simulink library "lib_SecCtrl_MASmsg"  (R2026a)
settings: Solver=VariableStepAuto
undefined symbols (not defined in the file): buses_lf, DiscIntNeverNeededParam, entity, iPs_lf, iQs_lf, last_send, m, Ps_lf, Qs_lf, set_DG_up, set_extra_satur, set_sending_cost, v_buses_mod
libraries: simulink x400, sl_discontinuities x10, eeGeneralControl x5
(part 12 of 12)

== system lib_SecCtrl_MASmsg/MAS messages/ID3/Send to neighbor1/one/select ==
  select : TriggerPort  TriggerType=function-call  IsSimulinkFunction=on  FunctionName=select  FunctionVisibility=scoped  VariantControl=(inherit)
  All : simulink/Logic and Bit Operations/Compare To Constant  relop===  const=0  OutDataTypeStr=boolean  ZeroCross=off
  Gain : Gain  OutDataTypeStr=double
  Gain2 : Gain  Gain=2  OutDataTypeStr=double
  Neighbor : simulink/Logic and Bit Operations/Compare To Constant  relop===  const=2  OutDataTypeStr=boolean  ZeroCross=off
  Sum : Sum  Inputs=|++
  u : ArgIn  DisableCoverage=on  ArgumentName=u
  y : ArgOut  ArgumentName=y
  wires:
  u/1 -> All/1, Neighbor/1
  Neighbor/1 -> Gain/1
  Gain2/1 -> Sum/2
  All/1 -> Gain2/1
  Sum/1 -> y/1
  Gain/1 -> Sum/1

== system lib_SecCtrl_MASmsg/MAS messages/ID3/Send to neighbor1/three/select ==
  select : TriggerPort  TriggerType=function-call  IsSimulinkFunction=on  FunctionName=select  FunctionVisibility=scoped  VariantControl=(inherit)
  All : simulink/Logic and Bit Operations/Compare To Constant  relop===  const=0  OutDataTypeStr=boolean  ZeroCross=off
  Gain : Gain  OutDataTypeStr=double
  Gain1 : Gain  Gain=2  OutDataTypeStr=double
  Gain2 : Gain  Gain=4  OutDataTypeStr=double
  Gain3 : Gain  Gain=3  OutDataTypeStr=double
  Neighbor1 : simulink/Logic and Bit Operations/Compare To Constant  relop===  const=0  OutDataTypeStr=boolean  ZeroCross=off
  Neighbor2 : simulink/Logic and Bit Operations/Compare To Constant  relop===  const=0  OutDataTypeStr=boolean  ZeroCross=off
  Neighbor3 : simulink/Logic and Bit Operations/Compare To Constant  relop===  const=0  OutDataTypeStr=boolean  ZeroCross=off
  Sum : Sum  Inputs=|++++
  u : ArgIn  DisableCoverage=on  ArgumentName=u
  y : ArgOut  ArgumentName=y
  wires:
  Neighbor2/1 -> Gain1/1
  u/1 -> Neighbor3/1, All/1, Neighbor1/1, Neighbor2/1
  Neighbor1/1 -> Gain/1
  Gain2/1 -> Sum/4
  All/1 -> Gain2/1
  Gain1/1 -> Sum/2
  Sum/1 -> y/1
  Gain/1 -> Sum/1
  Neighbor3/1 -> Gain3/1
  Gain3/1 -> Sum/3

== system lib_SecCtrl_MASmsg/MAS messages/ID3/Send to neighbor1/two/select ==
  select : TriggerPort  TriggerType=function-call  IsSimulinkFunction=on  FunctionName=select  FunctionVisibility=scoped  VariantControl=(inherit)
  All : simulink/Logic and Bit Operations/Compare To Constant  relop===  const=0  OutDataTypeStr=boolean  ZeroCross=off
  Gain : Gain  OutDataTypeStr=double
  Gain1 : Gain  Gain=2  OutDataTypeStr=double
  Gain2 : Gain  Gain=3  OutDataTypeStr=double
  Neighbor1 : simulink/Logic and Bit Operations/Compare To Constant  relop===  const=2  OutDataTypeStr=boolean  ZeroCross=off
  Neighbor2 : simulink/Logic and Bit Operations/Compare To Constant  relop===  const=4  OutDataTypeStr=boolean  ZeroCross=off
  Sum : Sum  Inputs=|+++
  u : ArgIn  DisableCoverage=on  ArgumentName=u
  y : ArgOut  ArgumentName=y
  wires:
  Neighbor2/1 -> Gain1/1
  u/1 -> All/1, Neighbor1/1, Neighbor2/1
  Neighbor1/1 -> Gain/1
  Gain2/1 -> Sum/3
  All/1 -> Gain2/1
  Gain1/1 -> Sum/2
  Sum/1 -> y/1
  Gain/1 -> Sum/1

== system lib_SecCtrl_MASmsg/MAS messages/ID3/Send to neighbor2/five/select ==
  select : TriggerPort  TriggerType=function-call  IsSimulinkFunction=on  FunctionName=select  FunctionVisibility=scoped  VariantControl=(inherit)
  All : simulink/Logic and Bit Operations/Compare To Constant  relop===  const=0  OutDataTypeStr=boolean  ZeroCross=off
  Gain : Gain  OutDataTypeStr=double
  Gain1 : Gain  Gain=2  OutDataTypeStr=double
  Gain2 : Gain  Gain=6  OutDataTypeStr=double
  Gain3 : Gain  Gain=3  OutDataTypeStr=double
  Gain4 : Gain  Gain=4  OutDataTypeStr=double
  Gain5 : Gain  Gain=5  OutDataTypeStr=double
  Neighbor1 : simulink/Logic and Bit Operations/Compare To Constant  relop===  const=2  OutDataTypeStr=boolean  ZeroCross=off
  Neighbor2 : simulink/Logic and Bit Operations/Compare To Constant  relop===  const=2  OutDataTypeStr=boolean  ZeroCross=off
  Neighbor3 : simulink/Logic and Bit Operations/Compare To Constant  relop===  const=0  OutDataTypeStr=boolean  ZeroCross=off
  Neighbor4 : simulink/Logic and Bit Operations/Compare To Constant  relop===  const=0  OutDataTypeStr=boolean  ZeroCross=off
  Neighbor5 : simulink/Logic and Bit Operations/Compare To Constant  relop===  const=0  OutDataTypeStr=boolean  ZeroCross=off
  Sum : Sum  Inputs=|++++++
  u : ArgIn  DisableCoverage=on  ArgumentName=u
  y : ArgOut  ArgumentName=y
  wires:
  Neighbor5/1 -> Gain5/1
  Gain5/1 -> Sum/5
  Neighbor2/1 -> Gain1/1
  u/1 -> Neighbor3/1, Neighbor4/1, All/1, Neighbor5/1, Neighbor1/1, Neighbor2/1
  Neighbor1/1 -> Gain/1
  Gain2/1 -> Sum/6
  All/1 -> Gain2/1
  Gain1/1 -> Sum/2
  Sum/1 -> y/1
  Gain/1 -> Sum/1
  Neighbor3/1 -> Gain3/1
  Gain3/1 -> Sum/3
  Gain4/1 -> Sum/4
  Neighbor4/1 -> Gain4/1

== system lib_SecCtrl_MASmsg/MAS messages/ID3/Send to neighbor2/four/select ==
  select : TriggerPort  TriggerType=function-call  IsSimulinkFunction=on  FunctionName=select  FunctionVisibility=scoped  VariantControl=(inherit)
  All : simulink/Logic and Bit Operations/Compare To Constant  relop===  const=0  OutDataTypeStr=boolean  ZeroCross=off
  Gain : Gain  OutDataTypeStr=double
  Gain1 : Gain  Gain=2  OutDataTypeStr=double
  Gain2 : Gain  Gain=5  OutDataTypeStr=double
  Gain3 : Gain  Gain=3  OutDataTypeStr=double
  Gain4 : Gain  Gain=4  OutDataTypeStr=double
  Neighbor1 : simulink/Logic and Bit Operations/Compare To Constant  relop===  const=1  OutDataTypeStr=boolean  ZeroCross=off
  Neighbor2 : simulink/Logic and Bit Operations/Compare To Constant  relop===  const=3  OutDataTypeStr=boolean  ZeroCross=off
  Neighbor3 : simulink/Logic and Bit Operations/Compare To Constant  relop===  const=0  OutDataTypeStr=boolean  ZeroCross=off
  Neighbor4 : simulink/Logic and Bit Operations/Compare To Constant  relop===  const=0  OutDataTypeStr=boolean  ZeroCross=off
  Sum : Sum  Inputs=|+++++
  u : ArgIn  DisableCoverage=on  ArgumentName=u
  y : ArgOut  ArgumentName=y
  wires:
  Neighbor4/1 -> Gain4/1
  Gain4/1 -> Sum/4
  Gain3/1 -> Sum/3
  Neighbor3/1 -> Gain3/1
  Gain/1 -> Sum/1
  Sum/1 -> y/1
  Gain1/1 -> Sum/2
  All/1 -> Gain2/1
  Gain2/1 -> Sum/5
  Neighbor1/1 -> Gain/1
  u/1 -> Neighbor2/1, Neighbor1/1, All/1, Neighbor4/1, Neighbor3/1
  Neighbor2/1 -> Gain1/1

== system lib_SecCtrl_MASmsg/MAS messages/ID3/Send to neighbor2/one/select ==
  select : TriggerPort  TriggerType=function-call  IsSimulinkFunction=on  FunctionName=select  FunctionVisibility=scoped  VariantControl=(inherit)
  All : simulink/Logic and Bit Operations/Compare To Constant  relop===  const=0  OutDataTypeStr=boolean  ZeroCross=off
  Gain : Gain  OutDataTypeStr=double
  Gain2 : Gain  Gain=2  OutDataTypeStr=double
  Neighbor : simulink/Logic and Bit Operations/Compare To Constant  relop===  const=2  OutDataTypeStr=boolean  ZeroCross=off
  Sum : Sum  Inputs=|++
  u : ArgIn  DisableCoverage=on  ArgumentName=u
  y : ArgOut  ArgumentName=y
  wires:
  Gain/1 -> Sum/1
  Sum/1 -> y/1
  All/1 -> Gain2/1
  Gain2/1 -> Sum/2
  Neighbor/1 -> Gain/1
  u/1 -> Neighbor/1, All/1

== system lib_SecCtrl_MASmsg/MAS messages/ID3/Send to neighbor2/three/select ==
  select : TriggerPort  TriggerType=function-call  IsSimulinkFunction=on  FunctionName=select  FunctionVisibility=scoped  VariantControl=(inherit)
  All : simulink/Logic and Bit Operations/Compare To Constant  relop===  const=0  OutDataTypeStr=boolean  ZeroCross=off
  Gain : Gain  OutDataTypeStr=double
  Gain1 : Gain  Gain=2  OutDataTypeStr=double
  Gain2 : Gain  Gain=4  OutDataTypeStr=double
  Gain3 : Gain  Gain=3  OutDataTypeStr=double
  Neighbor1 : simulink/Logic and Bit Operations/Compare To Constant  relop===  const=0  OutDataTypeStr=boolean  ZeroCross=off
  Neighbor2 : simulink/Logic and Bit Operations/Compare To Constant  relop===  const=0  OutDataTypeStr=boolean  ZeroCross=off
  Neighbor3 : simulink/Logic and Bit Operations/Compare To Constant  relop===  const=0  OutDataTypeStr=boolean  ZeroCross=off
  Sum : Sum  Inputs=|++++
  u : ArgIn  DisableCoverage=on  ArgumentName=u
  y : ArgOut  ArgumentName=y
  wires:
  Gain3/1 -> Sum/3
  Neighbor3/1 -> Gain3/1
  Gain/1 -> Sum/1
  Sum/1 -> y/1
  Gain1/1 -> Sum/2
  All/1 -> Gain2/1
  Gain2/1 -> Sum/4
  Neighbor1/1 -> Gain/1
  u/1 -> Neighbor2/1, Neighbor1/1, All/1, Neighbor3/1
  Neighbor2/1 -> Gain1/1

== system lib_SecCtrl_MASmsg/MAS messages/ID3/Send to neighbor2/two/select ==
  select : TriggerPort  TriggerType=function-call  IsSimulinkFunction=on  FunctionName=select  FunctionVisibility=scoped  VariantControl=(inherit)
  All : simulink/Logic and Bit Operations/Compare To Constant  relop===  const=0  OutDataTypeStr=boolean  ZeroCross=off
  Gain : Gain  OutDataTypeStr=double
  Gain1 : Gain  Gain=2  OutDataTypeStr=double
  Gain2 : Gain  Gain=3  OutDataTypeStr=double
  Neighbor1 : simulink/Logic and Bit Operations/Compare To Constant  relop===  const=2  OutDataTypeStr=boolean  ZeroCross=off
  Neighbor2 : simulink/Logic and Bit Operations/Compare To Constant  relop===  const=4  OutDataTypeStr=boolean  ZeroCross=off
  Sum : Sum  Inputs=|+++
  u : ArgIn  DisableCoverage=on  ArgumentName=u
  y : ArgOut  ArgumentName=y
  wires:
  Gain/1 -> Sum/1
  Sum/1 -> y/1
  Gain1/1 -> Sum/2
  All/1 -> Gain2/1
  Gain2/1 -> Sum/3
  Neighbor1/1 -> Gain/1
  u/1 -> Neighbor2/1, Neighbor1/1, All/1
  Neighbor2/1 -> Gain1/1

== system lib_SecCtrl_MASmsg/MAS messages/ID4/Send to neighbor/five/select ==
  select : TriggerPort  TriggerType=function-call  IsSimulinkFunction=on  FunctionName=select  FunctionVisibility=scoped  VariantControl=(inherit)
  All : simulink/Logic and Bit Operations/Compare To Constant  relop===  const=0  OutDataTypeStr=boolean  ZeroCross=off
  Gain : Gain  OutDataTypeStr=double
  Gain1 : Gain  Gain=2  OutDataTypeStr=double
  Gain2 : Gain  Gain=6  OutDataTypeStr=double
  Gain3 : Gain  Gain=3  OutDataTypeStr=double
  Gain4 : Gain  Gain=4  OutDataTypeStr=double
  Gain5 : Gain  Gain=5  OutDataTypeStr=double
  Neighbor1 : simulink/Logic and Bit Operations/Compare To Constant  relop===  const=2  OutDataTypeStr=boolean  ZeroCross=off
  Neighbor2 : simulink/Logic and Bit Operations/Compare To Constant  relop===  const=2  OutDataTypeStr=boolean  ZeroCross=off
  Neighbor3 : simulink/Logic and Bit Operations/Compare To Constant  relop===  const=0  OutDataTypeStr=boolean  ZeroCross=off
  Neighbor4 : simulink/Logic and Bit Operations/Compare To Constant  relop===  const=0  OutDataTypeStr=boolean  ZeroCross=off
  Neighbor5 : simulink/Logic and Bit Operations/Compare To Constant  relop===  const=0  OutDataTypeStr=boolean  ZeroCross=off
  Sum : Sum  Inputs=|++++++
  u : ArgIn  DisableCoverage=on  ArgumentName=u
  y : ArgOut  ArgumentName=y
  wires:
  Neighbor5/1 -> Gain5/1
  Gain5/1 -> Sum/5
  Neighbor2/1 -> Gain1/1
  u/1 -> Neighbor3/1, Neighbor4/1, All/1, Neighbor5/1, Neighbor1/1, Neighbor2/1
  Neighbor1/1 -> Gain/1
  Gain2/1 -> Sum/6
  All/1 -> Gain2/1
  Gain1/1 -> Sum/2
  Sum/1 -> y/1
  Gain/1 -> Sum/1
  Neighbor3/1 -> Gain3/1
  Gain3/1 -> Sum/3
  Gain4/1 -> Sum/4
  Neighbor4/1 -> Gain4/1

== system lib_SecCtrl_MASmsg/MAS messages/ID4/Send to neighbor/four/select ==
  select : TriggerPort  TriggerType=function-call  IsSimulinkFunction=on  FunctionName=select  FunctionVisibility=scoped  VariantControl=(inherit)
  All : simulink/Logic and Bit Operations/Compare To Constant  relop===  const=0  OutDataTypeStr=boolean  ZeroCross=off
  Gain : Gain  OutDataTypeStr=double
  Gain1 : Gain  Gain=2  OutDataTypeStr=double
  Gain2 : Gain  Gain=5  OutDataTypeStr=double
  Gain3 : Gain  Gain=3  OutDataTypeStr=double
  Gain4 : Gain  Gain=4  OutDataTypeStr=double
  Neighbor1 : simulink/Logic and Bit Operations/Compare To Constant  relop===  const=1  OutDataTypeStr=boolean  ZeroCross=off
  Neighbor2 : simulink/Logic and Bit Operations/Compare To Constant  relop===  const=3  OutDataTypeStr=boolean  ZeroCross=off
  Neighbor3 : simulink/Logic and Bit Operations/Compare To Constant  relop===  const=0  OutDataTypeStr=boolean  ZeroCross=off
  Neighbor4 : simulink/Logic and Bit Operations/Compare To Constant  relop===  const=0  OutDataTypeStr=boolean  ZeroCross=off
  Sum : Sum  Inputs=|+++++
  u : ArgIn  DisableCoverage=on  ArgumentName=u
  y : ArgOut  ArgumentName=y
  wires:
  Neighbor4/1 -> Gain4/1
  Gain4/1 -> Sum/4
  Gain3/1 -> Sum/3
  Neighbor3/1 -> Gain3/1
  Gain/1 -> Sum/1
  Sum/1 -> y/1
  Gain1/1 -> Sum/2
  All/1 -> Gain2/1
  Gain2/1 -> Sum/5
  Neighbor1/1 -> Gain/1
  u/1 -> Neighbor2/1, Neighbor1/1, All/1, Neighbor4/1, Neighbor3/1
  Neighbor2/1 -> Gain1/1

== system lib_SecCtrl_MASmsg/MAS messages/ID4/Send to neighbor/one/select ==
  select : TriggerPort  TriggerType=function-call  IsSimulinkFunction=on  FunctionName=select  FunctionVisibility=scoped  VariantControl=(inherit)
  All : simulink/Logic and Bit Operations/Compare To Constant  relop===  const=0  OutDataTypeStr=boolean  ZeroCross=off
  Gain : Gain  OutDataTypeStr=double
  Gain2 : Gain  Gain=2  OutDataTypeStr=double
  Neighbor : simulink/Logic and Bit Operations/Compare To Constant  relop===  const=2  OutDataTypeStr=boolean  ZeroCross=off
  Sum : Sum  Inputs=|++
  u : ArgIn  DisableCoverage=on  ArgumentName=u
  y : ArgOut  ArgumentName=y
  wires:
  Gain/1 -> Sum/1
  Sum/1 -> y/1
  All/1 -> Gain2/1
  Gain2/1 -> Sum/2
  Neighbor/1 -> Gain/1
  u/1 -> Neighbor/1, All/1

== system lib_SecCtrl_MASmsg/MAS messages/ID4/Send to neighbor/three/select ==
  select : TriggerPort  TriggerType=function-call  IsSimulinkFunction=on  FunctionName=select  FunctionVisibility=scoped  VariantControl=(inherit)
  All : simulink/Logic and Bit Operations/Compare To Constant  relop===  const=0  OutDataTypeStr=boolean  ZeroCross=off
  Gain : Gain  OutDataTypeStr=double
  Gain1 : Gain  Gain=2  OutDataTypeStr=double
  Gain2 : Gain  Gain=4  OutDataTypeStr=double
  Gain3 : Gain  Gain=3  OutDataTypeStr=double
  Neighbor1 : simulink/Logic and Bit Operations/Compare To Constant  relop===  const=0  OutDataTypeStr=boolean  ZeroCross=off
  Neighbor2 : simulink/Logic and Bit Operations/Compare To Constant  relop===  const=0  OutDataTypeStr=boolean  ZeroCross=off
  Neighbor3 : simulink/Logic and Bit Operations/Compare To Constant  relop===  const=0  OutDataTypeStr=boolean  ZeroCross=off
  Sum : Sum  Inputs=|++++
  u : ArgIn  DisableCoverage=on  ArgumentName=u
  y : ArgOut  ArgumentName=y
  wires:
  Gain3/1 -> Sum/3
  Neighbor3/1 -> Gain3/1
  Gain/1 -> Sum/1
  Sum/1 -> y/1
  Gain1/1 -> Sum/2
  All/1 -> Gain2/1
  Gain2/1 -> Sum/4
  Neighbor1/1 -> Gain/1
  u/1 -> Neighbor2/1, Neighbor1/1, All/1, Neighbor3/1
  Neighbor2/1 -> Gain1/1

== system lib_SecCtrl_MASmsg/MAS messages/ID4/Send to neighbor/two/select ==
  select : TriggerPort  TriggerType=function-call  IsSimulinkFunction=on  FunctionName=select  FunctionVisibility=scoped  VariantControl=(inherit)
  All : simulink/Logic and Bit Operations/Compare To Constant  relop===  const=0  OutDataTypeStr=boolean  ZeroCross=off
  Gain : Gain  OutDataTypeStr=double
  Gain1 : Gain  Gain=2  OutDataTypeStr=double
  Gain2 : Gain  Gain=3  OutDataTypeStr=double
  Neighbor1 : simulink/Logic and Bit Operations/Compare To Constant  relop===  const=3  OutDataTypeStr=boolean  ZeroCross=off
  Neighbor2 : simulink/Logic and Bit Operations/Compare To Constant  relop===  const=5  OutDataTypeStr=boolean  ZeroCross=off
  Sum : Sum  Inputs=|+++
  u : ArgIn  DisableCoverage=on  ArgumentName=u
  y : ArgOut  ArgumentName=y
  wires:
  Gain/1 -> Sum/1
  Sum/1 -> y/1
  Gain1/1 -> Sum/2
  All/1 -> Gain2/1
  Gain2/1 -> Sum/3
  Neighbor1/1 -> Gain/1
  u/1 -> Neighbor2/1, Neighbor1/1, All/1
  Neighbor2/1 -> Gain1/1

== system lib_SecCtrl_MASmsg/MAS messages/ID4/Send to neighbor1/five/select ==
  select : TriggerPort  TriggerType=function-call  IsSimulinkFunction=on  FunctionName=select  FunctionVisibility=scoped  VariantControl=(inherit)
  All : simulink/Logic and Bit Operations/Compare To Constant  relop===  const=0  OutDataTypeStr=boolean  ZeroCross=off
  Gain : Gain  OutDataTypeStr=double
  Gain1 : Gain  Gain=2  OutDataTypeStr=double
  Gain2 : Gain  Gain=6  OutDataTypeStr=double
  Gain3 : Gain  Gain=3  OutDataTypeStr=double
  Gain4 : Gain  Gain=4  OutDataTypeStr=double
  Gain5 : Gain  Gain=5  OutDataTypeStr=double
  Neighbor1 : simulink/Logic and Bit Operations/Compare To Constant  relop===  const=2  OutDataTypeStr=boolean  ZeroCross=off
  Neighbor2 : simulink/Logic and Bit Operations/Compare To Constant  relop===  const=2  OutDataTypeStr=boolean  ZeroCross=off
  Neighbor3 : simulink/Logic and Bit Operations/Compare To Constant  relop===  const=0  OutDataTypeStr=boolean  ZeroCross=off
  Neighbor4 : simulink/Logic and Bit Operations/Compare To Constant  relop===  const=0  OutDataTypeStr=boolean  ZeroCross=off
  Neighbor5 : simulink/Logic and Bit Operations/Compare To Constant  relop===  const=0  OutDataTypeStr=boolean  ZeroCross=off
  Sum : Sum  Inputs=|++++++
  u : ArgIn  DisableCoverage=on  ArgumentName=u
  y : ArgOut  ArgumentName=y
  wires:
  Neighbor4/1 -> Gain4/1
  Gain4/1 -> Sum/4
  Gain3/1 -> Sum/3
  Neighbor3/1 -> Gain3/1
  Gain/1 -> Sum/1
  Sum/1 -> y/1
  Gain1/1 -> Sum/2
  All/1 -> Gain2/1
  Gain2/1 -> Sum/6
  Neighbor1/1 -> Gain/1
  u/1 -> Neighbor2/1, Neighbor1/1, Neighbor5/1, All/1, Neighbor4/1, Neighbor3/1
  Neighbor2/1 -> Gain1/1
  Gain5/1 -> Sum/5
  Neighbor5/1 -> Gain5/1

== system lib_SecCtrl_MASmsg/MAS messages/ID4/Send to neighbor1/four/select ==
  select : TriggerPort  TriggerType=function-call  IsSimulinkFunction=on  FunctionName=select  FunctionVisibility=scoped  VariantControl=(inherit)
  All : simulink/Logic and Bit Operations/Compare To Constant  relop===  const=0  OutDataTypeStr=boolean  ZeroCross=off
  Gain : Gain  OutDataTypeStr=double
  Gain1 : Gain  Gain=2  OutDataTypeStr=double
  Gain2 : Gain  Gain=5  OutDataTypeStr=double
  Gain3 : Gain  Gain=3  OutDataTypeStr=double
  Gain4 : Gain  Gain=4  OutDataTypeStr=double
  Neighbor1 : simulink/Logic and Bit Operations/Compare To Constant  relop===  const=1  OutDataTypeStr=boolean  ZeroCross=off
  Neighbor2 : simulink/Logic and Bit Operations/Compare To Constant  relop===  const=3  OutDataTypeStr=boolean  ZeroCross=off
  Neighbor3 : simulink/Logic and Bit Operations/Compare To Constant  relop===  const=0  OutDataTypeStr=boolean  ZeroCross=off
  Neighbor4 : simulink/Logic and Bit Operations/Compare To Constant  relop===  const=0  OutDataTypeStr=boolean  ZeroCross=off
  Sum : Sum  Inputs=|+++++
  u : ArgIn  DisableCoverage=on  ArgumentName=u
  y : ArgOut  ArgumentName=y
  wires:
  Neighbor2/1 -> Gain1/1
  u/1 -> Neighbor3/1, Neighbor4/1, All/1, Neighbor1/1, Neighbor2/1
  Neighbor1/1 -> Gain/1
  Gain2/1 -> Sum/5
  All/1 -> Gain2/1
  Gain1/1 -> Sum/2
  Sum/1 -> y/1
  Gain/1 -> Sum/1
  Neighbor3/1 -> Gain3/1
  Gain3/1 -> Sum/3
  Gain4/1 -> Sum/4
  Neighbor4/1 -> Gain4/1

== system lib_SecCtrl_MASmsg/MAS messages/ID4/Send to neighbor1/one/select ==
  select : TriggerPort  TriggerType=function-call  IsSimulinkFunction=on  FunctionName=select  FunctionVisibility=scoped  VariantControl=(inherit)
  All : simulink/Logic and Bit Operations/Compare To Constant  relop===  const=0  OutDataTypeStr=boolean  ZeroCross=off
  Gain : Gain  OutDataTypeStr=double
  Gain2 : Gain  Gain=2  OutDataTypeStr=double
  Neighbor : simulink/Logic and Bit Operations/Compare To Constant  relop===  const=2  OutDataTypeStr=boolean  ZeroCross=off
  Sum : Sum  Inputs=|++
  u : ArgIn  DisableCoverage=on  ArgumentName=u
  y : ArgOut  ArgumentName=y
  wires:
  u/1 -> All/1, Neighbor/1
  Neighbor/1 -> Gain/1
  Gain2/1 -> Sum/2
  All/1 -> Gain2/1
  Sum/1 -> y/1
  Gain/1 -> Sum/1

== system lib_SecCtrl_MASmsg/MAS messages/ID4/Send to neighbor1/three/select ==
  select : TriggerPort  TriggerType=function-call  IsSimulinkFunction=on  FunctionName=select  FunctionVisibility=scoped  VariantControl=(inherit)
  All : simulink/Logic and Bit Operations/Compare To Constant  relop===  const=0  OutDataTypeStr=boolean  ZeroCross=off
  Gain : Gain  OutDataTypeStr=double
  Gain1 : Gain  Gain=2  OutDataTypeStr=double
  Gain2 : Gain  Gain=4  OutDataTypeStr=double
  Gain3 : Gain  Gain=3  OutDataTypeStr=double
  Neighbor1 : simulink/Logic and Bit Operations/Compare To Constant  relop===  const=0  OutDataTypeStr=boolean  ZeroCross=off
  Neighbor2 : simulink/Logic and Bit Operations/Compare To Constant  relop===  const=0  OutDataTypeStr=boolean  ZeroCross=off
  Neighbor3 : simulink/Logic and Bit Operations/Compare To Constant  relop===  const=0  OutDataTypeStr=boolean  ZeroCross=off
  Sum : Sum  Inputs=|++++
  u : ArgIn  DisableCoverage=on  ArgumentName=u
  y : ArgOut  ArgumentName=y
  wires:
  Neighbor2/1 -> Gain1/1
  u/1 -> Neighbor3/1, All/1, Neighbor1/1, Neighbor2/1
  Neighbor1/1 -> Gain/1
  Gain2/1 -> Sum/4
  All/1 -> Gain2/1
  Gain1/1 -> Sum/2
  Sum/1 -> y/1
  Gain/1 -> Sum/1
  Neighbor3/1 -> Gain3/1
  Gain3/1 -> Sum/3

== system lib_SecCtrl_MASmsg/MAS messages/ID4/Send to neighbor1/two/select ==
  select : TriggerPort  TriggerType=function-call  IsSimulinkFunction=on  FunctionName=select  FunctionVisibility=scoped  VariantControl=(inherit)
  All : simulink/Logic and Bit Operations/Compare To Constant  relop===  const=0  OutDataTypeStr=boolean  ZeroCross=off
  Gain : Gain  OutDataTypeStr=double
  Gain1 : Gain  Gain=2  OutDataTypeStr=double
  Gain2 : Gain  Gain=3  OutDataTypeStr=double
  Neighbor1 : simulink/Logic and Bit Operations/Compare To Constant  relop===  const=3  OutDataTypeStr=boolean  ZeroCross=off
  Neighbor2 : simulink/Logic and Bit Operations/Compare To Constant  relop===  const=5  OutDataTypeStr=boolean  ZeroCross=off
  Sum : Sum  Inputs=|+++
  u : ArgIn  DisableCoverage=on  ArgumentName=u
  y : ArgOut  ArgumentName=y
  wires:
  Neighbor2/1 -> Gain1/1
  u/1 -> All/1, Neighbor1/1, Neighbor2/1
  Neighbor1/1 -> Gain/1
  Gain2/1 -> Sum/3
  All/1 -> Gain2/1
  Gain1/1 -> Sum/2
  Sum/1 -> y/1
  Gain/1 -> Sum/1

== system lib_SecCtrl_MASmsg/MAS messages/ID4/Send to neighbor2/five/select ==
  select : TriggerPort  TriggerType=function-call  IsSimulinkFunction=on  FunctionName=select  FunctionVisibility=scoped  VariantControl=(inherit)
  All : simulink/Logic and Bit Operations/Compare To Constant  relop===  const=0  OutDataTypeStr=boolean  ZeroCross=off
  Gain : Gain  OutDataTypeStr=double
  Gain1 : Gain  Gain=2  OutDataTypeStr=double
  Gain2 : Gain  Gain=6  OutDataTypeStr=double
  Gain3 : Gain  Gain=3  OutDataTypeStr=double
  Gain4 : Gain  Gain=4  OutDataTypeStr=double
  Gain5 : Gain  Gain=5  OutDataTypeStr=double
  Neighbor1 : simulink/Logic and Bit Operations/Compare To Constant  relop===  const=2  OutDataTypeStr=boolean  ZeroCross=off
  Neighbor2 : simulink/Logic and Bit Operations/Compare To Constant  relop===  const=2  OutDataTypeStr=boolean  ZeroCross=off
  Neighbor3 : simulink/Logic and Bit Operations/Compare To Constant  relop===  const=0  OutDataTypeStr=boolean  ZeroCross=off
  Neighbor4 : simulink/Logic and Bit Operations/Compare To Constant  relop===  const=0  OutDataTypeStr=boolean  ZeroCross=off
  Neighbor5 : simulink/Logic and Bit Operations/Compare To Constant  relop===  const=0  OutDataTypeStr=boolean  ZeroCross=off
  Sum : Sum  Inputs=|++++++
  u : ArgIn  DisableCoverage=on  ArgumentName=u
  y : ArgOut  ArgumentName=y
  wires:
  Neighbor5/1 -> Gain5/1
  Gain5/1 -> Sum/5
  Neighbor2/1 -> Gain1/1
  u/1 -> Neighbor3/1, Neighbor4/1, All/1, Neighbor5/1, Neighbor1/1, Neighbor2/1
  Neighbor1/1 -> Gain/1
  Gain2/1 -> Sum/6
  All/1 -> Gain2/1
  Gain1/1 -> Sum/2
  Sum/1 -> y/1
  Gain/1 -> Sum/1
  Neighbor3/1 -> Gain3/1
  Gain3/1 -> Sum/3
  Gain4/1 -> Sum/4
  Neighbor4/1 -> Gain4/1

== system lib_SecCtrl_MASmsg/MAS messages/ID4/Send to neighbor2/four/select ==
  select : TriggerPort  TriggerType=function-call  IsSimulinkFunction=on  FunctionName=select  FunctionVisibility=scoped  VariantControl=(inherit)
  All : simulink/Logic and Bit Operations/Compare To Constant  relop===  const=0  OutDataTypeStr=boolean  ZeroCross=off
  Gain : Gain  OutDataTypeStr=double
  Gain1 : Gain  Gain=2  OutDataTypeStr=double
  Gain2 : Gain  Gain=5  OutDataTypeStr=double
  Gain3 : Gain  Gain=3  OutDataTypeStr=double
  Gain4 : Gain  Gain=4  OutDataTypeStr=double
  Neighbor1 : simulink/Logic and Bit Operations/Compare To Constant  relop===  const=1  OutDataTypeStr=boolean  ZeroCross=off
  Neighbor2 : simulink/Logic and Bit Operations/Compare To Constant  relop===  const=3  OutDataTypeStr=boolean  ZeroCross=off
  Neighbor3 : simulink/Logic and Bit Operations/Compare To Constant  relop===  const=0  OutDataTypeStr=boolean  ZeroCross=off
  Neighbor4 : simulink/Logic and Bit Operations/Compare To Constant  relop===  const=0  OutDataTypeStr=boolean  ZeroCross=off
  Sum : Sum  Inputs=|+++++
  u : ArgIn  DisableCoverage=on  ArgumentName=u
  y : ArgOut  ArgumentName=y
  wires:
  Neighbor4/1 -> Gain4/1
  Gain4/1 -> Sum/4
  Gain3/1 -> Sum/3
  Neighbor3/1 -> Gain3/1
  Gain/1 -> Sum/1
  Sum/1 -> y/1
  Gain1/1 -> Sum/2
  All/1 -> Gain2/1
  Gain2/1 -> Sum/5
  Neighbor1/1 -> Gain/1
  u/1 -> Neighbor2/1, Neighbor1/1, All/1, Neighbor4/1, Neighbor3/1
  Neighbor2/1 -> Gain1/1

== system lib_SecCtrl_MASmsg/MAS messages/ID4/Send to neighbor2/one/select ==
  select : TriggerPort  TriggerType=function-call  IsSimulinkFunction=on  FunctionName=select  FunctionVisibility=scoped  VariantControl=(inherit)
  All : simulink/Logic and Bit Operations/Compare To Constant  relop===  const=0  OutDataTypeStr=boolean  ZeroCross=off
  Gain : Gain  OutDataTypeStr=double
  Gain2 : Gain  Gain=2  OutDataTypeStr=double
  Neighbor : simulink/Logic and Bit Operations/Compare To Constant  relop===  const=2  OutDataTypeStr=boolean  ZeroCross=off
  Sum : Sum  Inputs=|++
  u : ArgIn  DisableCoverage=on  ArgumentName=u
  y : ArgOut  ArgumentName=y
  wires:
  Gain/1 -> Sum/1
  Sum/1 -> y/1
  All/1 -> Gain2/1
  Gain2/1 -> Sum/2
  Neighbor/1 -> Gain/1
  u/1 -> Neighbor/1, All/1

== system lib_SecCtrl_MASmsg/MAS messages/ID4/Send to neighbor2/three/select ==
  select : TriggerPort  TriggerType=function-call  IsSimulinkFunction=on  FunctionName=select  FunctionVisibility=scoped  VariantControl=(inherit)
  All : simulink/Logic and Bit Operations/Compare To Constant  relop===  const=0  OutDataTypeStr=boolean  ZeroCross=off
  Gain : Gain  OutDataTypeStr=double
  Gain1 : Gain  Gain=2  OutDataTypeStr=double
  Gain2 : Gain  Gain=4  OutDataTypeStr=double
  Gain3 : Gain  Gain=3  OutDataTypeStr=double
  Neighbor1 : simulink/Logic and Bit Operations/Compare To Constant  relop===  const=0  OutDataTypeStr=boolean  ZeroCross=off
  Neighbor2 : simulink/Logic and Bit Operations/Compare To Constant  relop===  const=0  OutDataTypeStr=boolean  ZeroCross=off
  Neighbor3 : simulink/Logic and Bit Operations/Compare To Constant  relop===  const=0  OutDataTypeStr=boolean  ZeroCross=off
  Sum : Sum  Inputs=|++++
  u : ArgIn  DisableCoverage=on  ArgumentName=u
  y : ArgOut  ArgumentName=y
  wires:
  Gain3/1 -> Sum/3
  Neighbor3/1 -> Gain3/1
  Gain/1 -> Sum/1
  Sum/1 -> y/1
  Gain1/1 -> Sum/2
  All/1 -> Gain2/1
  Gain2/1 -> Sum/4
  Neighbor1/1 -> Gain/1
  u/1 -> Neighbor2/1, Neighbor1/1, All/1, Neighbor3/1
  Neighbor2/1 -> Gain1/1

== system lib_SecCtrl_MASmsg/MAS messages/ID4/Send to neighbor2/two/select ==
  select : TriggerPort  TriggerType=function-call  IsSimulinkFunction=on  FunctionName=select  FunctionVisibility=scoped  VariantControl=(inherit)
  All : simulink/Logic and Bit Operations/Compare To Constant  relop===  const=0  OutDataTypeStr=boolean  ZeroCross=off
  Gain : Gain  OutDataTypeStr=double
  Gain1 : Gain  Gain=2  OutDataTypeStr=double
  Gain2 : Gain  Gain=3  OutDataTypeStr=double
  Neighbor1 : simulink/Logic and Bit Operations/Compare To Constant  relop===  const=3  OutDataTypeStr=boolean  ZeroCross=off
  Neighbor2 : simulink/Logic and Bit Operations/Compare To Constant  relop===  const=5  OutDataTypeStr=boolean  ZeroCross=off
  Sum : Sum  Inputs=|+++
  u : ArgIn  DisableCoverage=on  ArgumentName=u
  y : ArgOut  ArgumentName=y
  wires:
  Gain/1 -> Sum/1
  Sum/1 -> y/1
  Gain1/1 -> Sum/2
  All/1 -> Gain2/1
  Gain2/1 -> Sum/3
  Neighbor1/1 -> Gain/1
  u/1 -> Neighbor2/1, Neighbor1/1, All/1
  Neighbor2/1 -> Gain1/1

== system lib_SecCtrl_MASmsg/MAS messages/ID5/Send to neighbor/five/select ==
  select : TriggerPort  TriggerType=function-call  IsSimulinkFunction=on  FunctionName=select  FunctionVisibility=scoped  VariantControl=(inherit)
  All : simulink/Logic and Bit Operations/Compare To Constant  relop===  const=0  OutDataTypeStr=boolean  ZeroCross=off
  Gain : Gain  OutDataTypeStr=double
  Gain1 : Gain  Gain=2  OutDataTypeStr=double
  Gain2 : Gain  Gain=6  OutDataTypeStr=double
  Gain3 : Gain  Gain=3  OutDataTypeStr=double
  Gain4 : Gain  Gain=4  OutDataTypeStr=double
  Gain5 : Gain  Gain=5  OutDataTypeStr=double
  Neighbor1 : simulink/Logic and Bit Operations/Compare To Constant  relop===  const=2  OutDataTypeStr=boolean  ZeroCross=off
  Neighbor2 : simulink/Logic and Bit Operations/Compare To Constant  relop===  const=2  OutDataTypeStr=boolean  ZeroCross=off
  Neighbor3 : simulink/Logic and Bit Operations/Compare To Constant  relop===  const=0  OutDataTypeStr=boolean  ZeroCross=off
  Neighbor4 : simulink/Logic and Bit Operations/Compare To Constant  relop===  const=0  OutDataTypeStr=boolean  ZeroCross=off
  Neighbor5 : simulink/Logic and Bit Operations/Compare To Constant  relop===  const=0  OutDataTypeStr=boolean  ZeroCross=off
  Sum : Sum  Inputs=|++++++
  u : ArgIn  DisableCoverage=on  ArgumentName=u
  y : ArgOut  ArgumentName=y
  wires:
  Neighbor5/1 -> Gain5/1
  Gain5/1 -> Sum/5
  Neighbor2/1 -> Gain1/1
  u/1 -> Neighbor3/1, Neighbor4/1, All/1, Neighbor5/1, Neighbor1/1, Neighbor2/1
  Neighbor1/1 -> Gain/1
  Gain2/1 -> Sum/6
  All/1 -> Gain2/1
  Gain1/1 -> Sum/2
  Sum/1 -> y/1
  Gain/1 -> Sum/1
  Neighbor3/1 -> Gain3/1
  Gain3/1 -> Sum/3
  Gain4/1 -> Sum/4
  Neighbor4/1 -> Gain4/1

== system lib_SecCtrl_MASmsg/MAS messages/ID5/Send to neighbor/four/select ==
  select : TriggerPort  TriggerType=function-call  IsSimulinkFunction=on  FunctionName=select  FunctionVisibility=scoped  VariantControl=(inherit)
  All : simulink/Logic and Bit Operations/Compare To Constant  relop===  const=0  OutDataTypeStr=boolean  ZeroCross=off
  Gain : Gain  OutDataTypeStr=double
  Gain1 : Gain  Gain=2  OutDataTypeStr=double
  Gain2 : Gain  Gain=5  OutDataTypeStr=double
  Gain3 : Gain  Gain=3  OutDataTypeStr=double
  Gain4 : Gain  Gain=4  OutDataTypeStr=double
  Neighbor1 : simulink/Logic and Bit Operations/Compare To Constant  relop===  const=1  OutDataTypeStr=boolean  ZeroCross=off
  Neighbor2 : simulink/Logic and Bit Operations/Compare To Constant  relop===  const=3  OutDataTypeStr=boolean  ZeroCross=off
  Neighbor3 : simulink/Logic and Bit Operations/Compare To Constant  relop===  const=0  OutDataTypeStr=boolean  ZeroCross=off
  Neighbor4 : simulink/Logic and Bit Operations/Compare To Constant  relop===  const=0  OutDataTypeStr=boolean  ZeroCross=off
  Sum : Sum  Inputs=|+++++
  u : ArgIn  DisableCoverage=on  ArgumentName=u
  y : ArgOut  ArgumentName=y
  wires:
  Neighbor4/1 -> Gain4/1
  Gain4/1 -> Sum/4
  Gain3/1 -> Sum/3
  Neighbor3/1 -> Gain3/1
  Gain/1 -> Sum/1
  Sum/1 -> y/1
  Gain1/1 -> Sum/2
  All/1 -> Gain2/1
  Gain2/1 -> Sum/5
  Neighbor1/1 -> Gain/1
  u/1 -> Neighbor2/1, Neighbor1/1, All/1, Neighbor4/1, Neighbor3/1
  Neighbor2/1 -> Gain1/1

== system lib_SecCtrl_MASmsg/MAS messages/ID5/Send to neighbor/one/select ==
  select : TriggerPort  TriggerType=function-call  IsSimulinkFunction=on  FunctionName=select  FunctionVisibility=scoped  VariantControl=(inherit)
  All : simulink/Logic and Bit Operations/Compare To Constant  relop===  const=0  OutDataTypeStr=boolean  ZeroCross=off
  Gain : Gain  OutDataTypeStr=double
  Gain2 : Gain  Gain=2  OutDataTypeStr=double
  Neighbor : simulink/Logic and Bit Operations/Compare To Constant  relop===  const=2  OutDataTypeStr=boolean  ZeroCross=off
  Sum : Sum  Inputs=|++
  u : ArgIn  DisableCoverage=on  ArgumentName=u
  y : ArgOut  ArgumentName=y
  wires:
  Gain/1 -> Sum/1
  Sum/1 -> y/1
  All/1 -> Gain2/1
  Gain2/1 -> Sum/2
  Neighbor/1 -> Gain/1
  u/1 -> Neighbor/1, All/1

== system lib_SecCtrl_MASmsg/MAS messages/ID5/Send to neighbor/three/select ==
  select : TriggerPort  TriggerType=function-call  IsSimulinkFunction=on  FunctionName=select  FunctionVisibility=scoped  VariantControl=(inherit)
  All : simulink/Logic and Bit Operations/Compare To Constant  relop===  const=0  OutDataTypeStr=boolean  ZeroCross=off
  Gain : Gain  OutDataTypeStr=double
  Gain1 : Gain  Gain=2  OutDataTypeStr=double
  Gain2 : Gain  Gain=4  OutDataTypeStr=double
  Gain3 : Gain  Gain=3  OutDataTypeStr=double
  Neighbor1 : simulink/Logic and Bit Operations/Compare To Constant  relop===  const=0  OutDataTypeStr=boolean  ZeroCross=off
  Neighbor2 : simulink/Logic and Bit Operations/Compare To Constant  relop===  const=0  OutDataTypeStr=boolean  ZeroCross=off
  Neighbor3 : simulink/Logic and Bit Operations/Compare To Constant  relop===  const=0  OutDataTypeStr=boolean  ZeroCross=off
  Sum : Sum  Inputs=|++++
  u : ArgIn  DisableCoverage=on  ArgumentName=u
  y : ArgOut  ArgumentName=y
  wires:
  Gain3/1 -> Sum/3
  Neighbor3/1 -> Gain3/1
  Gain/1 -> Sum/1
  Sum/1 -> y/1
  Gain1/1 -> Sum/2
  All/1 -> Gain2/1
  Gain2/1 -> Sum/4
  Neighbor1/1 -> Gain/1
  u/1 -> Neighbor2/1, Neighbor1/1, All/1, Neighbor3/1
  Neighbor2/1 -> Gain1/1

== system lib_SecCtrl_MASmsg/MAS messages/ID5/Send to neighbor/two/select ==
  select : TriggerPort  TriggerType=function-call  IsSimulinkFunction=on  FunctionName=select  FunctionVisibility=scoped  VariantControl=(inherit)
  All : simulink/Logic and Bit Operations/Compare To Constant  relop===  const=0  OutDataTypeStr=boolean  ZeroCross=off
  Gain : Gain  OutDataTypeStr=double
  Gain1 : Gain  Gain=2  OutDataTypeStr=double
  Gain2 : Gain  Gain=3  OutDataTypeStr=double
  Neighbor1 : simulink/Logic and Bit Operations/Compare To Constant  relop===  const=4  OutDataTypeStr=boolean  ZeroCross=off
  Neighbor2 : simulink/Logic and Bit Operations/Compare To Constant  relop===  const=1  OutDataTypeStr=boolean  ZeroCross=off
  Sum : Sum  Inputs=|+++
  u : ArgIn  DisableCoverage=on  ArgumentName=u
  y : ArgOut  ArgumentName=y
  wires:
  Gain/1 -> Sum/1
  Sum/1 -> y/1
  Gain1/1 -> Sum/2
  All/1 -> Gain2/1
  Gain2/1 -> Sum/3
  Neighbor1/1 -> Gain/1
  u/1 -> Neighbor2/1, Neighbor1/1, All/1
  Neighbor2/1 -> Gain1/1

== system lib_SecCtrl_MASmsg/MAS messages/ID5/Send to neighbor1/five/select ==
  select : TriggerPort  TriggerType=function-call  IsSimulinkFunction=on  FunctionName=select  FunctionVisibility=scoped  VariantControl=(inherit)
  All : simulink/Logic and Bit Operations/Compare To Constant  relop===  const=0  OutDataTypeStr=boolean  ZeroCross=off
  Gain : Gain  OutDataTypeStr=double
  Gain1 : Gain  Gain=2  OutDataTypeStr=double
  Gain2 : Gain  Gain=6  OutDataTypeStr=double
  Gain3 : Gain  Gain=3  OutDataTypeStr=double
  Gain4 : Gain  Gain=4  OutDataTypeStr=double
  Gain5 : Gain  Gain=5  OutDataTypeStr=double
  Neighbor1 : simulink/Logic and Bit Operations/Compare To Constant  relop===  const=2  OutDataTypeStr=boolean  ZeroCross=off
  Neighbor2 : simulink/Logic and Bit Operations/Compare To Constant  relop===  const=2  OutDataTypeStr=boolean  ZeroCross=off
  Neighbor3 : simulink/Logic and Bit Operations/Compare To Constant  relop===  const=0  OutDataTypeStr=boolean  ZeroCross=off
  Neighbor4 : simulink/Logic and Bit Operations/Compare To Constant  relop===  const=0  OutDataTypeStr=boolean  ZeroCross=off
  Neighbor5 : simulink/Logic and Bit Operations/Compare To Constant  relop===  const=0  OutDataTypeStr=boolean  ZeroCross=off
  Sum : Sum  Inputs=|++++++
  u : ArgIn  DisableCoverage=on  ArgumentName=u
  y : ArgOut  ArgumentName=y
  wires:
  Neighbor4/1 -> Gain4/1
  Gain4/1 -> Sum/4
  Gain3/1 -> Sum/3
  Neighbor3/1 -> Gain3/1
  Gain/1 -> Sum/1
  Sum/1 -> y/1
  Gain1/1 -> Sum/2
  All/1 -> Gain2/1
  Gain2/1 -> Sum/6
  Neighbor1/1 -> Gain/1
  u/1 -> Neighbor2/1, Neighbor1/1, Neighbor5/1, All/1, Neighbor4/1, Neighbor3/1
  Neighbor2/1 -> Gain1/1
  Gain5/1 -> Sum/5
  Neighbor5/1 -> Gain5/1

== system lib_SecCtrl_MASmsg/MAS messages/ID5/Send to neighbor1/four/select ==
  select : TriggerPort  TriggerType=function-call  IsSimulinkFunction=on  FunctionName=select  FunctionVisibility=scoped  VariantControl=(inherit)
  All : simulink/Logic and Bit Operations/Compare To Constant  relop===  const=0  OutDataTypeStr=boolean  ZeroCross=off
  Gain : Gain  OutDataTypeStr=double
  Gain1 : Gain  Gain=2  OutDataTypeStr=double
  Gain2 : Gain  Gain=5  OutDataTypeStr=double
  Gain3 : Gain  Gain=3  OutDataTypeStr=double
  Gain4 : Gain  Gain=4  OutDataTypeStr=double
  Neighbor1 : simulink/Logic and Bit Operations/Compare To Constant  relop===  const=1  OutDataTypeStr=boolean  ZeroCross=off
  Neighbor2 : simulink/Logic and Bit Operations/Compare To Constant  relop===  const=3  OutDataTypeStr=boolean  ZeroCross=off
  Neighbor3 : simulink/Logic and Bit Operations/Compare To Constant  relop===  const=0  OutDataTypeStr=boolean  ZeroCross=off
  Neighbor4 : simulink/Logic and Bit Operations/Compare To Constant  relop===  const=0  OutDataTypeStr=boolean  ZeroCross=off
  Sum : Sum  Inputs=|+++++
  u : ArgIn  DisableCoverage=on  ArgumentName=u
  y : ArgOut  ArgumentName=y
  wires:
  Neighbor2/1 -> Gain1/1
  u/1 -> Neighbor3/1, Neighbor4/1, All/1, Neighbor1/1, Neighbor2/1
  Neighbor1/1 -> Gain/1
  Gain2/1 -> Sum/5
  All/1 -> Gain2/1
  Gain1/1 -> Sum/2
  Sum/1 -> y/1
  Gain/1 -> Sum/1
  Neighbor3/1 -> Gain3/1
  Gain3/1 -> Sum/3
  Gain4/1 -> Sum/4
  Neighbor4/1 -> Gain4/1

== system lib_SecCtrl_MASmsg/MAS messages/ID5/Send to neighbor1/one/select ==
  select : TriggerPort  TriggerType=function-call  IsSimulinkFunction=on  FunctionName=select  FunctionVisibility=scoped  VariantControl=(inherit)
  All : simulink/Logic and Bit Operations/Compare To Constant  relop===  const=0  OutDataTypeStr=boolean  ZeroCross=off
  Gain : Gain  OutDataTypeStr=double
  Gain2 : Gain  Gain=2  OutDataTypeStr=double
  Neighbor : simulink/Logic and Bit Operations/Compare To Constant  relop===  const=2  OutDataTypeStr=boolean  ZeroCross=off
  Sum : Sum  Inputs=|++
  u : ArgIn  DisableCoverage=on  ArgumentName=u
  y : ArgOut  ArgumentName=y
  wires:
  u/1 -> All/1, Neighbor/1
  Neighbor/1 -> Gain/1
  Gain2/1 -> Sum/2
  All/1 -> Gain2/1
  Sum/1 -> y/1
  Gain/1 -> Sum/1

== system lib_SecCtrl_MASmsg/MAS messages/ID5/Send to neighbor1/three/select ==
  select : TriggerPort  TriggerType=function-call  IsSimulinkFunction=on  FunctionName=select  FunctionVisibility=scoped  VariantControl=(inherit)
  All : simulink/Logic and Bit Operations/Compare To Constant  relop===  const=0  OutDataTypeStr=boolean  ZeroCross=off
  Gain : Gain  OutDataTypeStr=double
  Gain1 : Gain  Gain=2  OutDataTypeStr=double
  Gain2 : Gain  Gain=4  OutDataTypeStr=double
  Gain3 : Gain  Gain=3  OutDataTypeStr=double
  Neighbor1 : simulink/Logic and Bit Operations/Compare To Constant  relop===  const=0  OutDataTypeStr=boolean  ZeroCross=off
  Neighbor2 : simulink/Logic and Bit Operations/Compare To Constant  relop===  const=0  OutDataTypeStr=boolean  ZeroCross=off
  Neighbor3 : simulink/Logic and Bit Operations/Compare To Constant  relop===  const=0  OutDataTypeStr=boolean  ZeroCross=off
  Sum : Sum  Inputs=|++++
  u : ArgIn  DisableCoverage=on  ArgumentName=u
  y : ArgOut  ArgumentName=y
  wires:
  Neighbor2/1 -> Gain1/1
  u/1 -> Neighbor3/1, All/1, Neighbor1/1, Neighbor2/1
  Neighbor1/1 -> Gain/1
  Gain2/1 -> Sum/4
  All/1 -> Gain2/1
  Gain1/1 -> Sum/2
  Sum/1 -> y/1
  Gain/1 -> Sum/1
  Neighbor3/1 -> Gain3/1
  Gain3/1 -> Sum/3

== system lib_SecCtrl_MASmsg/MAS messages/ID5/Send to neighbor1/two/select ==
  select : TriggerPort  TriggerType=function-call  IsSimulinkFunction=on  FunctionName=select  FunctionVisibility=scoped  VariantControl=(inherit)
  All : simulink/Logic and Bit Operations/Compare To Constant  relop===  const=0  OutDataTypeStr=boolean  ZeroCross=off
  Gain : Gain  OutDataTypeStr=double
  Gain1 : Gain  Gain=2  OutDataTypeStr=double
  Gain2 : Gain  Gain=3  OutDataTypeStr=double
  Neighbor1 : simulink/Logic and Bit Operations/Compare To Constant  relop===  const=4  OutDataTypeStr=boolean  ZeroCross=off
  Neighbor2 : simulink/Logic and Bit Operations/Compare To Constant  relop===  const=1  OutDataTypeStr=boolean  ZeroCross=off
  Sum : Sum  Inputs=|+++
  u : ArgIn  DisableCoverage=on  ArgumentName=u
  y : ArgOut  ArgumentName=y
  wires:
  Neighbor2/1 -> Gain1/1
  u/1 -> All/1, Neighbor1/1, Neighbor2/1
  Neighbor1/1 -> Gain/1
  Gain2/1 -> Sum/3
  All/1 -> Gain2/1
  Gain1/1 -> Sum/2
  Sum/1 -> y/1
  Gain/1 -> Sum/1

== system lib_SecCtrl_MASmsg/MAS messages/ID5/Send to neighbor2/five/select ==
  select : TriggerPort  TriggerType=function-call  IsSimulinkFunction=on  FunctionName=select  FunctionVisibility=scoped  VariantControl=(inherit)
  All : simulink/Logic and Bit Operations/Compare To Constant  relop===  const=0  OutDataTypeStr=boolean  ZeroCross=off
  Gain : Gain  OutDataTypeStr=double
  Gain1 : Gain  Gain=2  OutDataTypeStr=double
  Gain2 : Gain  Gain=6  OutDataTypeStr=double
  Gain3 : Gain  Gain=3  OutDataTypeStr=double
  Gain4 : Gain  Gain=4  OutDataTypeStr=double
  Gain5 : Gain  Gain=5  OutDataTypeStr=double
  Neighbor1 : simulink/Logic and Bit Operations/Compare To Constant  relop===  const=2  OutDataTypeStr=boolean  ZeroCross=off
  Neighbor2 : simulink/Logic and Bit Operations/Compare To Constant  relop===  const=2  OutDataTypeStr=boolean  ZeroCross=off
  Neighbor3 : simulink/Logic and Bit Operations/Compare To Constant  relop===  const=0  OutDataTypeStr=boolean  ZeroCross=off
  Neighbor4 : simulink/Logic and Bit Operations/Compare To Constant  relop===  const=0  OutDataTypeStr=boolean  ZeroCross=off
  Neighbor5 : simulink/Logic and Bit Operations/Compare To Constant  relop===  const=0  OutDataTypeStr=boolean  ZeroCross=off
  Sum : Sum  Inputs=|++++++
  u : ArgIn  DisableCoverage=on  ArgumentName=u
  y : ArgOut  ArgumentName=y
  wires:
  Neighbor5/1 -> Gain5/1
  Gain5/1 -> Sum/5
  Neighbor2/1 -> Gain1/1
  u/1 -> Neighbor3/1, Neighbor4/1, All/1, Neighbor5/1, Neighbor1/1, Neighbor2/1
  Neighbor1/1 -> Gain/1
  Gain2/1 -> Sum/6
  All/1 -> Gain2/1
  Gain1/1 -> Sum/2
  Sum/1 -> y/1
  Gain/1 -> Sum/1
  Neighbor3/1 -> Gain3/1
  Gain3/1 -> Sum/3
  Gain4/1 -> Sum/4
  Neighbor4/1 -> Gain4/1

== system lib_SecCtrl_MASmsg/MAS messages/ID5/Send to neighbor2/four/select ==
  select : TriggerPort  TriggerType=function-call  IsSimulinkFunction=on  FunctionName=select  FunctionVisibility=scoped  VariantControl=(inherit)
  All : simulink/Logic and Bit Operations/Compare To Constant  relop===  const=0  OutDataTypeStr=boolean  ZeroCross=off
  Gain : Gain  OutDataTypeStr=double
  Gain1 : Gain  Gain=2  OutDataTypeStr=double
  Gain2 : Gain  Gain=5  OutDataTypeStr=double
  Gain3 : Gain  Gain=3  OutDataTypeStr=double
  Gain4 : Gain  Gain=4  OutDataTypeStr=double
  Neighbor1 : simulink/Logic and Bit Operations/Compare To Constant  relop===  const=1  OutDataTypeStr=boolean  ZeroCross=off
  Neighbor2 : simulink/Logic and Bit Operations/Compare To Constant  relop===  const=3  OutDataTypeStr=boolean  ZeroCross=off
  Neighbor3 : simulink/Logic and Bit Operations/Compare To Constant  relop===  const=0  OutDataTypeStr=boolean  ZeroCross=off
  Neighbor4 : simulink/Logic and Bit Operations/Compare To Constant  relop===  const=0  OutDataTypeStr=boolean  ZeroCross=off
  Sum : Sum  Inputs=|+++++
  u : ArgIn  DisableCoverage=on  ArgumentName=u
  y : ArgOut  ArgumentName=y
  wires:
  Neighbor4/1 -> Gain4/1
  Gain4/1 -> Sum/4
  Gain3/1 -> Sum/3
  Neighbor3/1 -> Gain3/1
  Gain/1 -> Sum/1
  Sum/1 -> y/1
  Gain1/1 -> Sum/2
  All/1 -> Gain2/1
  Gain2/1 -> Sum/5
  Neighbor1/1 -> Gain/1
  u/1 -> Neighbor2/1, Neighbor1/1, All/1, Neighbor4/1, Neighbor3/1
  Neighbor2/1 -> Gain1/1

== system lib_SecCtrl_MASmsg/MAS messages/ID5/Send to neighbor2/one/select ==
  select : TriggerPort  TriggerType=function-call  IsSimulinkFunction=on  FunctionName=select  FunctionVisibility=scoped  VariantControl=(inherit)
  All : simulink/Logic and Bit Operations/Compare To Constant  relop===  const=0  OutDataTypeStr=boolean  ZeroCross=off
  Gain : Gain  OutDataTypeStr=double
  Gain2 : Gain  Gain=2  OutDataTypeStr=double
  Neighbor : simulink/Logic and Bit Operations/Compare To Constant  relop===  const=2  OutDataTypeStr=boolean  ZeroCross=off
  Sum : Sum  Inputs=|++
  u : ArgIn  DisableCoverage=on  ArgumentName=u
  y : ArgOut  ArgumentName=y
  wires:
  Gain/1 -> Sum/1
  Sum/1 -> y/1
  All/1 -> Gain2/1
  Gain2/1 -> Sum/2
  Neighbor/1 -> Gain/1
  u/1 -> Neighbor/1, All/1

== system lib_SecCtrl_MASmsg/MAS messages/ID5/Send to neighbor2/three/select ==
  select : TriggerPort  TriggerType=function-call  IsSimulinkFunction=on  FunctionName=select  FunctionVisibility=scoped  VariantControl=(inherit)
  All : simulink/Logic and Bit Operations/Compare To Constant  relop===  const=0  OutDataTypeStr=boolean  ZeroCross=off
  Gain : Gain  OutDataTypeStr=double
  Gain1 : Gain  Gain=2  OutDataTypeStr=double
  Gain2 : Gain  Gain=4  OutDataTypeStr=double
  Gain3 : Gain  Gain=3  OutDataTypeStr=double
  Neighbor1 : simulink/Logic and Bit Operations/Compare To Constant  relop===  const=0  OutDataTypeStr=boolean  ZeroCross=off
  Neighbor2 : simulink/Logic and Bit Operations/Compare To Constant  relop===  const=0  OutDataTypeStr=boolean  ZeroCross=off
  Neighbor3 : simulink/Logic and Bit Operations/Compare To Constant  relop===  const=0  OutDataTypeStr=boolean  ZeroCross=off
  Sum : Sum  Inputs=|++++
  u : ArgIn  DisableCoverage=on  ArgumentName=u
  y : ArgOut  ArgumentName=y
  wires:
  Gain3/1 -> Sum/3
  Neighbor3/1 -> Gain3/1
  Gain/1 -> Sum/1
  Sum/1 -> y/1
  Gain1/1 -> Sum/2
  All/1 -> Gain2/1
  Gain2/1 -> Sum/4
  Neighbor1/1 -> Gain/1
  u/1 -> Neighbor2/1, Neighbor1/1, All/1, Neighbor3/1
  Neighbor2/1 -> Gain1/1

== system lib_SecCtrl_MASmsg/MAS messages/ID5/Send to neighbor2/two/select ==
  select : TriggerPort  TriggerType=function-call  IsSimulinkFunction=on  FunctionName=select  FunctionVisibility=scoped  VariantControl=(inherit)
  All : simulink/Logic and Bit Operations/Compare To Constant  relop===  const=0  OutDataTypeStr=boolean  ZeroCross=off
  Gain : Gain  OutDataTypeStr=double
  Gain1 : Gain  Gain=2  OutDataTypeStr=double
  Gain2 : Gain  Gain=3  OutDataTypeStr=double
  Neighbor1 : simulink/Logic and Bit Operations/Compare To Constant  relop===  const=4  OutDataTypeStr=boolean  ZeroCross=off
  Neighbor2 : simulink/Logic and Bit Operations/Compare To Constant  relop===  const=1  OutDataTypeStr=boolean  ZeroCross=off
  Sum : Sum  Inputs=|+++
  u : ArgIn  DisableCoverage=on  ArgumentName=u
  y : ArgOut  ArgumentName=y
  wires:
  Gain/1 -> Sum/1
  Sum/1 -> y/1
  Gain1/1 -> Sum/2
  All/1 -> Gain2/1
  Gain2/1 -> Sum/3
  Neighbor1/1 -> Gain/1
  u/1 -> Neighbor2/1, Neighbor1/1, All/1
  Neighbor2/1 -> Gain1/1
